simulink model "uC_Stateflow_after"  (Simulink 7.7)
settings: Solver=FixedStepDiscrete  SolverMode=SingleTasking  StartTime=0  StopTime=10.0  FixedStep=0.001  RelTol=1e-3
InitFcn:
  | St=0.01;
  | idleSPL=170;
  | idleSPR=170;
  | deltaIdle=80;
libraries: simulink x18, dsPICdrivers x7
settings Model: Creator=AKS1DY  LastModifiedBy=pcadmin
settings OptimizationCC: OptimizeModelRefInitCode=on  LifeSpan=1
settings HardwareCC: ProdBitPerInt=16  ProdBitPerPointer=16  ProdEndianess=LittleEndian  ProdWordSize=16  ProdHWDeviceType=16-bit Generic
settings RTWCC: SystemTargetFile=dspic.tlc  MakeCommand=make_CreateMPLAB  TemplateMakefile=dspic_pic30_gcc.tmf  PostCodeGenCommand=dsPIC_Compile()  Description=Embedded Target for Microchip dsPIC (real-time)  ProcessScript=dspic_make_rtw_hook
settings CodeAppCC: IgnoreCustomStorageClasses=off
settings STFCustomTargetCC: FunctionExecutionProfile=off  IncludeMdlTerminateFcn=off  CombineOutputUpdateFcns=on  SuppressErrorStatus=on  ERTCustomFileBanners=on  SupportContinuousTime=off  SupportNonInlinedSFcns=off  SystemTargetFile=dspic.tlc
settings ERTTargetCC: FunctionExecutionProfile=off  MultiwordLength=2048  ParMdlRefBuildCompliant=off  CompOptLevelCompliant=off  IncludeMdlTerminateFcn=off  SuppressErrorStatus=on  ERTFirstTimeCompliant=off  ModelStepFunctionPrototypeControlCompliant=off  CPPClassGenCompliant=off  ExtModeMexFile=ext_serial_win32_comm  InlinedParameterPlacement=NonHierarchical  ERTSrcFileBannerTemplate=dsPIC_code_template.cgt  ERTHdrFileBannerTemplate=dsPIC_code_template.cgt  ERTDataSrcFileTemplate=dsPIC_code_template.cgt  ERTDataHdrFileTemplate=dsPIC_code_template.cgt  ERTCustomFileTemplate=dsPIC_main.tlc  ConvertIfToSwitch=off
settings CustomProperty: DataType=string  Value=C:\PROGRA~1\MATLAB\R2011a\bin\win32\gmake

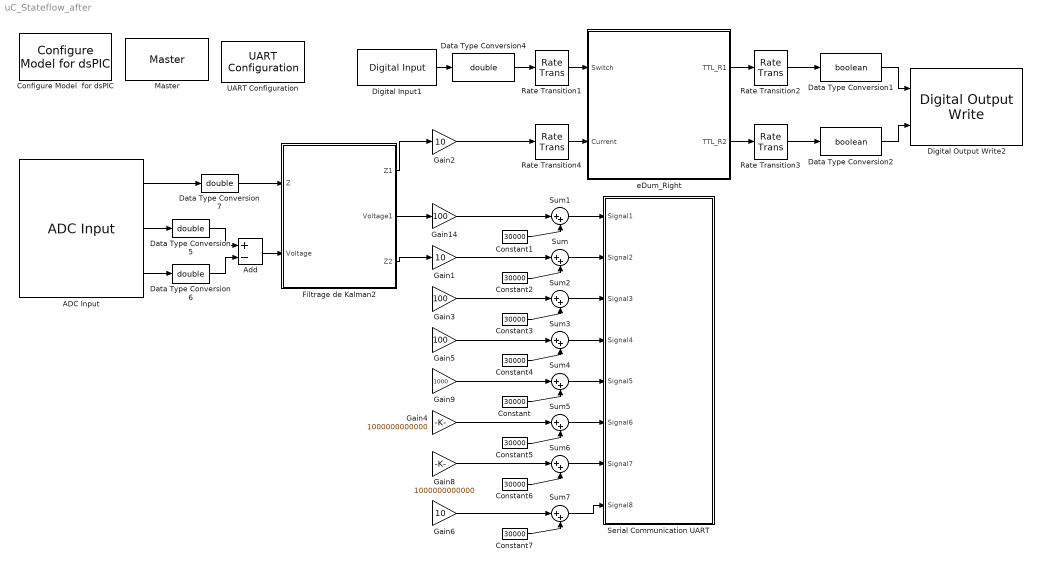
== system uC_Stateflow_after ==
  ADC Input : dsPICdrivers/Peripheral I//O/ADC Input  Tag=dsPIC_ADC  Priority=5  ADC_TYPE=12 bits  ADC_MODE=Continuous sampling & get last channel value  NbrSampleStep=1  VoltRefpopup="AVdd  -  AVss"  OutFormatBitspopup=0000 dddd dddd dddd : Integer  InterruptPriority=6  ANCHANNELS=[1 8 9]  MaxName=ANmax = 4095  Rin=1e2  ADCS=53  SAMC=1  Temperature=25  DMAChannel=0  SampleTime=St  Status="OK  |  Tsmp=6.750e-007 |  T/Channel=1.012e-005 |  Tall=3.037e-005"  SSRC=auto convert
  Add : Sum  Inputs=+-
  Configure Model  for dsPIC : dsPICdrivers/Simulink Configuration/Configure Model  for dsPIC
  Constant{,1..7} (8 alike) : Constant  Value=30000  SampleTime=St
  Data Type Conversion1 : DataTypeConversion  OutDataTypeStr=boolean
  Data Type Conversion2 : DataTypeConversion  OutDataTypeStr=boolean
  Data Type Conversion{4..7} (4 alike) : DataTypeConversion  OutDataTypeStr=double
  Digital Input1 : dsPICdrivers/Digital I//O/Digital Input  Tag=dsPIC_Digital_Input  PORT=D  Pin=[2]  SampleTime=St  OrderingInOutPopup=None
  Digital Output Write2 : dsPICdrivers/Digital I//O/Digital Output Write  Tag=dsPIC_Digital_Output  Priority=5  PORT=A  Pin=[6 7]  Simultaneous=on  OrderingInOutPopup=None
  Filtrage de Kalman2 : Stateflow chart  TreatAsAtomicUnit=on
  Gain1 : Gain  Gain=10
  Gain14 : Gain  Gain=100
  Gain2 : Gain  Gain=10
  Gain3 : Gain  Gain=100
  Gain4 : Gain  Gain=1000000000000
  Gain5 : Gain  Gain=100
  Gain6 : Gain  Gain=10
  Gain8 : Gain  Gain=1000000000000
  Gain9 : Gain  Gain=1000
  Master : dsPICdrivers/Master  Tag=dsPIC_MASTER  Priority=1  TimeStepType=Free Run  picType=33fJ256MC710a  fcy=40000000  Quartz_33f=8e6  PLLActive_33f=on  fcyDesired_33f=40E6  tmr1="[1  39999  0]"  tmr1Info="Time Step : 0.001  ;   Error : 0%  PR1=39999"  tmr2345="[0  0  0  0  0  0  0  0]"  tmr2345cfg=[-1 -1 -1 -1 -1 -1 -1 -1]  IOautoConf=on  typePort="[ 0   0   0   0   0   0  10  10   0   0   0   0   0   0   0   0   0   8   9   0   0   0   0   0   8   8   0   0   0   0   0   0   0   0   0   0   0   0   0   0   0   0   0   0   0   0   0   0   0   0   9   0   0   0   0   0   0   0   0   0   0   0   0   0   0   0   0   0   0   0   0   0   0   0   0   0   0   0   0   0   0   0   0   0   4   5   0   0   0   0   0   0   0   0   0   0   0   0   0   0   0   0   0   0   0   0   0   0   0   0   0   0 ]"  TRIS="[ 65343  65535  65535  65535  65535  65535  65535 ]"  ADPCFG=12582916  MasterBusyPort=None  MasterOverloadPort=None  FOSC=Quartz (XT - HS)  ClockSwitchMonitor=Both disabled  TempProtection_33f=TEMP_ON  FPBOR=<empty>  PWRT=disable  MCLR=<empty>  ICD=ICS_PGD1  JTAGEN=JTAGEN_OFF  PowerSave=off  OverrideFcy=off  NewFcy=1e6  PR2345="[65535  65535  65535  65535  65535  65535  65535  65535]"
  Rate Transition1 : RateTransition  OutPortSampleTime=0.01
  Rate Transition2 : RateTransition  OutPortSampleTime=St
  Rate Transition3 : RateTransition  OutPortSampleTime=St
  Rate Transition4 : RateTransition  OutPortSampleTime=0.01
  Serial Communication UART : Subsystem  Description=Send data from microcontroleur to computer
  Sum{,1..7} (8 alike) : Sum  Inputs=|++
  UART Configuration : dsPICdrivers/Serial PORT/UART Configuration  Tag=dsPIC_config_UART  Priority=2  UART=2  proposed_BAUD=Custom  BAUD=128000  ALT_TX_RX=off  InterruptTxWhen=When Transmit Buffer is empty  TXInterruptPri=1  TxBufferSize=1024  TXEN=on  InterruptRxWhen=When Receive Buffer is full (contain 4 characters)  RXInterruptPri=2  RxBufferSize=1024  DoNotImplementRxInterrupt=off  DoNotImplementTxInterrupt=off  UxBRG=19  Info="UxBRG = 19   ||  Real Baud : 125000   ||  % error : -2.3438  ||  max 12.5 Bytes / Step"  RealBaud=0  ERROR=-2.3438  BYTES_STEP=12.5
  eDum_Right : Stateflow chart  TreatAsAtomicUnit=on
  wires:
  Digital Input1/1 -> Data Type Conversion4/1
  Data Type Conversion4/1 -> Rate Transition1/1
  Data Type Conversion1/1 -> Digital Output Write2/1
  Data Type Conversion2/1 -> Digital Output Write2/2
  eDum_Right/1(TTL_R1) -> Rate Transition2/1
  ADC Input/1 -> Data Type Conversion7/1
  Data Type Conversion7/1 -> Filtrage de Kalman2/1(Z)
  ADC Input/2 -> Data Type Conversion5/1
  ADC Input/3 -> Data Type Conversion6/1
  Data Type Conversion5/1 -> Add/1
  Data Type Conversion6/1 -> Add/2
  Add/1 -> Filtrage de Kalman2/2(Voltage)
  Gain1/1 -> Sum/1
  Sum/1 -> Serial Communication UART/2(Signal2)
  Sum1/1 -> Serial Communication UART/1(Signal1)
  Sum4/1 -> Serial Communication UART/5(Signal5)
  Constant1/1 -> Sum1/2
  Constant2/1 -> Sum/2
  Constant/1 -> Sum4/2
  Filtrage de Kalman2/1(Z1) -> Gain2/1
  Gain2/1 -> Rate Transition4/1
  Gain3/1 -> Sum2/1
  Constant3/1 -> Sum2/2
  Sum2/1 -> Serial Communication UART/3(Signal3)
  Gain5/1 -> Sum3/1
  Constant4/1 -> Sum3/2
  Sum3/1 -> Serial Communication UART/4(Signal4)
  Constant5/1 -> Sum5/2
  Sum5/1 -> Serial Communication UART/6(Signal6)
  Constant6/1 -> Sum6/2
  Sum6/1 -> Serial Communication UART/7(Signal7)
  Constant7/1 -> Sum7/2
  Sum7/1 -> Serial Communication UART/8(Signal8)
  eDum_Right/2(TTL_R2) -> Rate Transition3/1
  Gain9/1 -> Sum4/1
  Gain8/1 -> Sum6/1
  Gain4/1 -> Sum5/1
  Gain6/1 -> Sum7/1
  Gain14/1 -> Sum1/1
  Rate Transition1/1 -> eDum_Right/1(Switch)
  Rate Transition4/1 -> eDum_Right/2(Current)
  Rate Transition2/1 -> Data Type Conversion1/1
  Rate Transition3/1 -> Data Type Conversion2/1
  Filtrage de Kalman2/2(Voltage1) -> Gain14/1
  Filtrage de Kalman2/3(Z2) -> Gain1/1

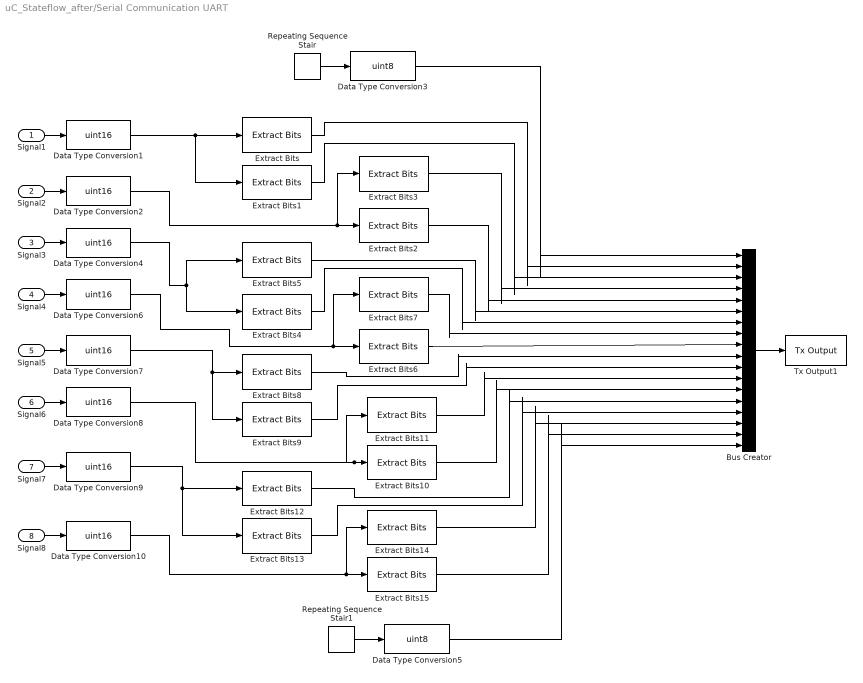
== system uC_Stateflow_after/Serial Communication UART ==
  Signal1 : Inport
  Signal2 : Inport  Port=2
  Signal3 : Inport  Port=3
  Signal4 : Inport  Port=4
  Signal5 : Inport  Port=5
  Signal6 : Inport  Port=6
  Signal7 : Inport  Port=7
  Signal8 : Inport  Port=8
  Bus Creator : BusCreator  Inputs=18
  Data Type Conversion{1..2,4,6..10} (8 alike) : DataTypeConversion  OutDataTypeStr=uint16  RndMeth=Ceiling
  Data Type Conversion3 : DataTypeConversion  OutDataTypeStr=uint8
  Data Type Conversion5 : DataTypeConversion  OutDataTypeStr=uint8
  Extract Bits{,3,5,7..8,11..12,14} (8 alike) : simulink/Logic and Bit Operations/Extract Bits  SystemSampleTime=-1  bitsToExtract=Range of bits  numBits=8  bitIdxRange=[8 15]  outScalingMode=Treat bit field as an integer
  Extract Bits{1..2,4,6,9..10,13,15} (8 alike) : simulink/Logic and Bit Operations/Extract Bits  SystemSampleTime=-1  bitsToExtract=Lower half  numBits=8  bitIdxRange=[0 7]  outScalingMode=Preserve fixed-point scaling
  Repeating Sequence Stair : simulink/Sources/Repeating Sequence Stair  SystemSampleTime=-1  OutValues=[2 4 1].'  tsamp=-1  OutMin=[]  OutMax=[]  OutDataTypeStr=double  OutputDataTypeScalingMode=double  OutDataType=fixdt(0,8)  ConRadixGroup=Best Precision: Vector-wise  OutScaling=2^-12
  Repeating Sequence Stair1 : simulink/Sources/Repeating Sequence Stair  SystemSampleTime=-1  OutValues=[3 3 3].'  tsamp=-1  OutMin=[]  OutMax=[]  OutDataTypeStr=double  OutputDataTypeScalingMode=double  OutDataType=fixdt(0,8)  ConRadixGroup=Best Precision: Vector-wise  OutScaling=2^-12
  Tx Output1 : dsPICdrivers/Serial PORT/Tx Output  Tag=dsPIC_TX  Priority=5  UART=2  OrderingInOutPopup=None
  wires:
  Data Type Conversion1/1 -> Extract Bits/1, Extract Bits1/1
  Bus Creator/1 -> Tx Output1/1
  Extract Bits/1 -> Bus Creator/2
  Extract Bits1/1 -> Bus Creator/3
  Repeating Sequence Stair/1 -> Data Type Conversion3/1
  Data Type Conversion3/1 -> Bus Creator/1
  Repeating Sequence Stair1/1 -> Data Type Conversion5/1
  Data Type Conversion5/1 -> Bus Creator/18
  Data Type Conversion2/1 -> Extract Bits3/1, Extract Bits2/1
  Data Type Conversion4/1 -> Extract Bits5/1, Extract Bits4/1
  Extract Bits5/1 -> Bus Creator/6
  Extract Bits4/1 -> Bus Creator/7
  Extract Bits3/1 -> Bus Creator/4
  Extract Bits2/1 -> Bus Creator/5
  Extract Bits7/1 -> Bus Creator/8
  Extract Bits6/1 -> Bus Creator/9
  Data Type Conversion6/1 -> Extract Bits7/1, Extract Bits6/1
  Data Type Conversion7/1 -> Extract Bits8/1, Extract Bits9/1
  Extract Bits8/1 -> Bus Creator/10
  Extract Bits9/1 -> Bus Creator/11
  Data Type Conversion8/1 -> Extract Bits11/1, Extract Bits10/1
  Extract Bits11/1 -> Bus Creator/12
  Extract Bits10/1 -> Bus Creator/13
  Data Type Conversion9/1 -> Extract Bits12/1, Extract Bits13/1
  Extract Bits12/1 -> Bus Creator/14
  Extract Bits13/1 -> Bus Creator/15
  Data Type Conversion10/1 -> Extract Bits14/1, Extract Bits15/1
  Extract Bits14/1 -> Bus Creator/16
  Extract Bits15/1 -> Bus Creator/17
  Signal1/1 -> Data Type Conversion1/1
  Signal2/1 -> Data Type Conversion2/1
  Signal3/1 -> Data Type Conversion4/1
  Signal4/1 -> Data Type Conversion6/1
  Signal5/1 -> Data Type Conversion7/1
  Signal6/1 -> Data Type Conversion8/1
  Signal7/1 -> Data Type Conversion9/1
  Signal8/1 -> Data Type Conversion10/1

== matlab function Filtrage de Kalman2 ==
  data: Z1 output double; Voltage1 output double; Z2 output double; Z input double; Voltage input double
function [Z1,Voltage1,Z2] = fcn(Z,Voltage)


Voltage=(Voltage*0.004);
Voltage1=Voltage;
Z=(50/12412)*Z;
if Voltage<=-0.3
    Z=-Z;
else
end
Z1=Z;
Z2=Z;

== stateflow chart eDum_Right ==
  settings: updateMethod=DISCRETE  sampleTime=0.01
  state Clockwise1
    entry: TTL_R1=1;
    TTL_R2=1;
  state Counterclockwise1
    entry: TTL_R1=1;
    TTL_R2=0;
  state Break3
    entry: TTL_R1=0;
    TTL_R2=0;
  state Break1
    entry: TTL_R1=0;
    TTL_R2=0;
  Break1 -> Counterclockwise1 : [after(10,tick) && Switch==1]
  (default) -> Break1
  Counterclockwise1 -> Break3 : [after(300,tick) || (Current>=100 && after(20,tick))]
  Break3 -> ? : [after(10,tick) && Switch==1]
  Clockwise1 -> Break1 : [after(200,tick)]
  data: Switch input uint8; TTL_R1 output double; TTL_R2 output double; Current input double
